simulink model "can2_mcu_odom_unpack"  (R2026b)
settings: Solver=VariableStepAuto
libraries: svdutilitieslib x1
settings Model: Creator=aomar  LastModifiedBy=aomar

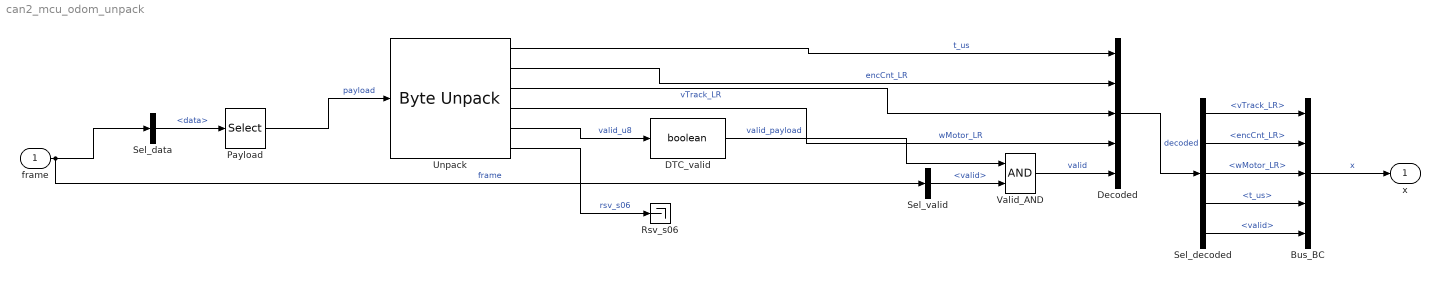
== system can2_mcu_odom_unpack ==
  frame : Inport  OutDataTypeStr=Bus: Bus_CanFrame64
  Bus_BC : BusCreator  Inputs=5  OutDataTypeStr=Bus: Bus_OdomMeas  NonVirtualBus=on
      settings: InheritFromInputs=off
  DTC_valid : DataTypeConversion  OutDataTypeStr=boolean  SaturateOnIntegerOverflow=off  RndMeth=Floor
  Decoded : BusCreator  Inputs=5
  Payload : Selector  InputPortWidth=64  IndexOptions=Index vector (dialog)  Indices=1:32  OutputSizes=1
  Rsv_s06 : Terminator
  Sel_data : BusSelector  OutputSignals=data
  Sel_decoded : BusSelector  OutputSignals=vTrack_LR,encCnt_LR,wMotor_LR,t_us,valid
  Sel_valid : BusSelector  OutputSignals=valid
  Unpack : svdutilitieslib/Byte Unpack  dimensions={1,2,2,2,1,3}  datatypes={'uint32','int32','single','single','uint8','uint8'}  byteAlign=1  blockPlatform=arduinoert
      settings: LibrarySourceBlock=mcblib/Signal Management/Byte Unpack
  Valid_AND : Logic  AllPortsSameDT=off  OutDataTypeStr=boolean
  x : Outport  OutDataTypeStr=Bus: Bus_OdomMeas
  wires:
  frame/1 -> Sel_data/1, Sel_valid/1  "frame"
  Sel_data/1 -> Payload/1  "<data>"
  Payload/1 -> Unpack/1  "payload"
  Unpack/1 -> Decoded/1  "t_us"
  Unpack/2 -> Decoded/2  "encCnt_LR"
  Unpack/3 -> Decoded/3  "vTrack_LR"
  Unpack/4 -> Decoded/4  "wMotor_LR"
  Unpack/5 -> DTC_valid/1  "valid_u8"
  Unpack/6 -> Rsv_s06/1  "rsv_s06"
  DTC_valid/1 -> Valid_AND/1  "valid_payload"
  Sel_valid/1 -> Valid_AND/2  "<valid>"
  Valid_AND/1 -> Decoded/5  "valid"
  Decoded/1 -> Sel_decoded/1  "decoded"
  Sel_decoded/1 -> Bus_BC/1  "<vTrack_LR>"
  Sel_decoded/2 -> Bus_BC/2  "<encCnt_LR>"
  Sel_decoded/3 -> Bus_BC/3  "<wMotor_LR>"
  Sel_decoded/4 -> Bus_BC/4  "<t_us>"
  Sel_decoded/5 -> Bus_BC/5  "<valid>"
  Bus_BC/1 -> x/1  "x"
